simulink model "solar_hydrogen_microgrid"  (R2026a)
settings: Solver=ode4  StopTime=86400  FixedStep=1
settings Model: Creator=rabbu  LastModifiedBy=rabbu

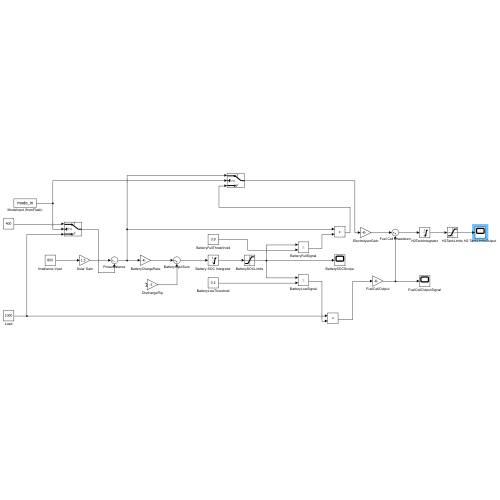
[thumbnail: Simulink's stored preview of the top-level diagram]
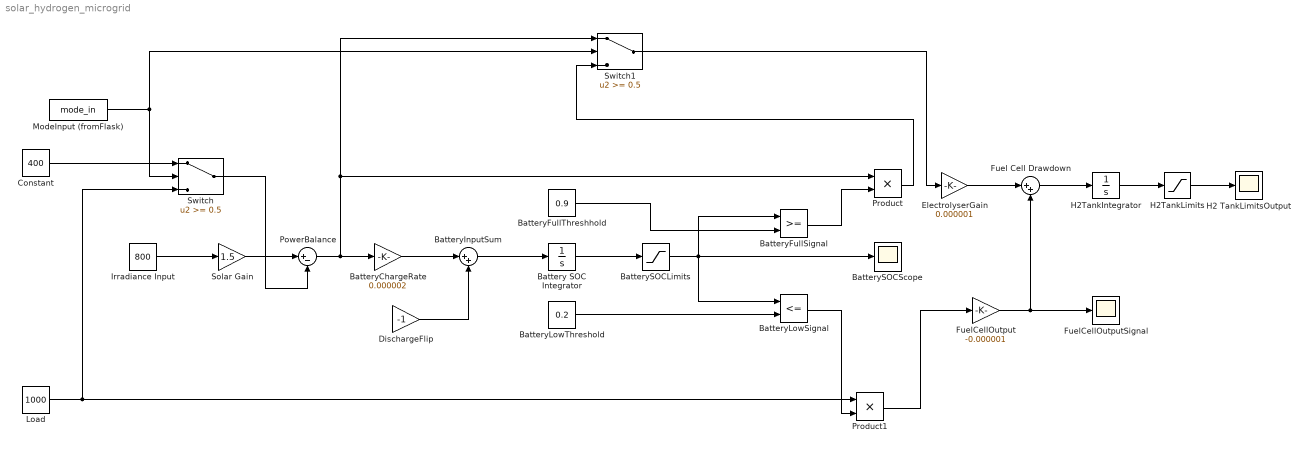
== system solar_hydrogen_microgrid ==
  Battery SOC Integrator : Integrator  InitialCondition=0.5  LimitOutput=on  UpperSaturationLimit=1  LowerSaturationLimit=0
  BatteryChargeRate : Gain  Gain=0.000002
  BatteryFullSignal : RelationalOperator  OutDataTypeStr=boolean  RndMeth=Simplest  InputSameDT=off
  BatteryFullThreshhold : Constant  Value=0.9
  BatteryInputSum : Sum  Inputs=|++
  BatteryLowSignal : RelationalOperator  Operator=<=  OutDataTypeStr=boolean  RndMeth=Simplest  InputSameDT=off
  BatteryLowThreshold : Constant  Value=0.2
  BatterySOCLimits : Saturate  UpperLimit=1  LowerLimit=0
  BatterySOCScope : Scope
      settings: ActiveDisplayYMinimum=0.22765950598392654  ActiveDisplayYMaximum=0.99971853144189848
  Constant : Constant  Value=400
  DischargeFlip : Gain  Gain=-1
  ElectrolyserGain : Gain  Gain=0.000001
  Fuel Cell Drawdown : Sum  Inputs=|++
  FuelCellOutput : Gain  Gain=-0.000001
  FuelCellOutputSignal : Scope
      settings: ActiveDisplayYMinimum=-0.0024395556113320904  ActiveDisplayYMaximum=0.0012285461995505547  DataLoggingVariableName=ScopeData2
  H2 TankLimitsOutput : Scope
      settings: ActiveDisplayYMinimum=-0.47940491640752381  ActiveDisplayYMaximum=1.6400727192461955
  H2TankIntegrator : Integrator  InitialCondition=0.5  LimitOutput=on  UpperSaturationLimit=1  LowerSaturationLimit=0
  H2TankLimits : Saturate  UpperLimit=1  LowerLimit=0
  Irradiance Input : Constant  Value=800
  Load : Constant  Value=1000
  ModeInput (fromFlask) : FromWorkspace  VariableName=mode_in  OutputAfterFinalValue=Holding final value
  PowerBalance : Sum  Inputs=|+-
  Product : Product
  Product1 : Product
  Solar Gain : Gain  Gain=1.5
  Switch : Switch  Threshold=0.5  SaturateOnIntegerOverflow=off  InputSameDT=off
  Switch1 : Switch  Threshold=0.5  SaturateOnIntegerOverflow=off  InputSameDT=off
  wires:
  Irradiance Input/1 -> Solar Gain/1
  Solar Gain/1 -> PowerBalance/1
  Load/1 -> Switch/3, Product1/1
  PowerBalance/1 -> BatteryChargeRate/1, Switch1/1, Product/1
  Battery SOC Integrator/1 -> BatterySOCLimits/1
  BatterySOCLimits/1 -> BatterySOCScope/1, BatteryLowSignal/1, BatteryFullSignal/1
  BatteryLowThreshold/1 -> BatteryLowSignal/2
  BatteryFullThreshhold/1 -> BatteryFullSignal/2
  BatteryChargeRate/1 -> BatteryInputSum/1
  BatteryInputSum/1 -> Battery SOC Integrator/1
  DischargeFlip/1 -> BatteryInputSum/2
  BatteryFullSignal/1 -> Product/2
  ElectrolyserGain/1 -> Fuel Cell Drawdown/1
  H2TankIntegrator/1 -> H2TankLimits/1
  H2TankLimits/1 -> H2 TankLimitsOutput/1
  BatteryLowSignal/1 -> Product1/2
  Product1/1 -> FuelCellOutput/1
  FuelCellOutput/1 -> Fuel Cell Drawdown/2, FuelCellOutputSignal/1
  Fuel Cell Drawdown/1 -> H2TankIntegrator/1
  ModeInput (fromFlask)/1 -> Switch1/2, Switch/2
  Switch/1 -> PowerBalance/2
  Product/1 -> Switch1/3
  Switch1/1 -> ElectrolyserGain/1
  Constant/1 -> Switch/1
